simulink model "FluxObserverTest"  (R2026b)
settings: Solver=FixedStepDiscrete  StopTime=fluxTestCfg.Duration  FixedStep=fluxCfg.Ts
PostLoadFcn:
  | addpath(fullfile(fileparts(get_param(bdroot,'FileName')),'..','build_process'));initialize_flux_test(bdroot);
model workspace (MAT data in the model file):
  fluxCfg.Ts = 5e-05
  fluxCfg.Rs = 0.5
  fluxCfg.L = 0.001
  fluxCfg.Flux = 0.035
  fluxCfg.PolePairs = 4
  fluxCfg.LeakEnable = 1
  fluxCfg.LeakHz = 10
  fluxCfg.DcEnable = 1
  fluxCfg.DcHz = 3
  fluxCfg.FrequencyHz = 5
  fluxCfg.MinCompOmega = 20
  fluxCfg.FullCompOmega = 100
  fluxCfg.MaxCompGain = 4
  fluxCfg.MinFlux = 0.015
  fluxCfg.MaxFlux = 0.0525
  fluxCfg.MinOmega = 120
  fluxCfg.MaxResidual = 5
  fluxCfg.LeakA = 0.996863336985
  fluxCfg.LeakB = 4.99215423658e-05
  fluxCfg.DcA = 0.999057966197
  fluxCfg.FrequencyA = 0.998430436728
  fluxTestCfg.Duration = 1
  fluxTestCfg.ElectricalSpeed = 200
  fluxTestCfg.InitialAngle = 0.4
  fluxTestCfg.Id = -2
  fluxTestCfg.Iq = 2
  fluxTestCfg.Enable = 1
  fluxTestCfg.Reset = 0
  pllCfg.Ts = 5e-05
  pllCfg.NaturalFrequency = 40
  pllCfg.Damping = 0.707
  pllCfg.Kp = 355.376960974
  pllCfg.Ki = 63165.468167
  pllCfg.Kaw = 502.654824574
  pllCfg.OmegaMax = 1500
  pllCfg.MinMagnitude = 0.015
  pllCfg.LockError = 0.12
  pllCfg.LockSamples = 100
  pllCfg.Theta0 = 0
  pllCfg.Omega0 = 0
  testStim.time = []
  testStim.signals.values = [-4.24906479315 -4.31340004462 -4.37730395969 -4.44077014801 -4.50379226301 -4.56636400254 -4.62847910947 -4.69013137235 -4.75131462601 -4.81202275215 -4.87224968004 -4.93198938701 ... (180009 elements, 20001x9)]
  testStim.signals.dimensions = 9
libraries: FluxObserver x1
settings Model: Creator=24322  LastModifiedBy=24322

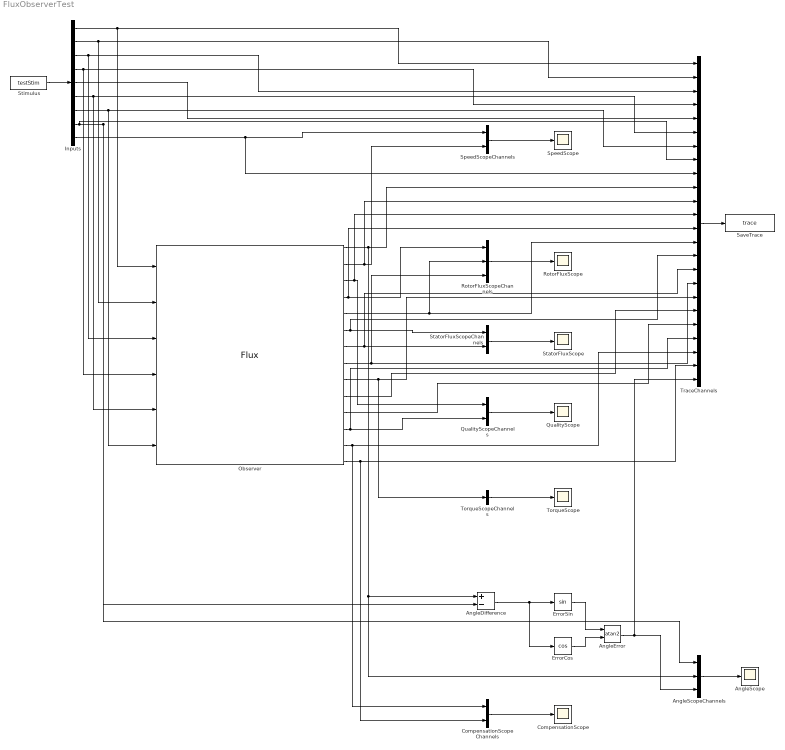
== system FluxObserverTest ==
  AngleDifference : Sum  Inputs=+-
  AngleError : Trigonometry  Operator=atan2
  AngleScope : Scope
  AngleScopeChannels : Mux  Inputs=3
  CompensationScope : Scope
  CompensationScopeChannels : Mux  Inputs=2
  ErrorCos : Trigonometry  Operator=cos
  ErrorSin : Trigonometry
  Inputs : Demux  Outputs=9
  Observer : FluxObserver/Flux  cfg=fluxCfg  trackerCfg=pllCfg
  QualityScope : Scope
  QualityScopeChannels : Mux  Inputs=2
  RotorFluxScope : Scope
  RotorFluxScopeChannels : Mux  Inputs=3
  SaveTrace : ToWorkspace  VariableName=trace  SaveFormat=Structure With Time  SampleTime=-1
  SpeedScope : Scope
  SpeedScopeChannels : Mux  Inputs=2
  StatorFluxScope : Scope
  StatorFluxScopeChannels : Mux  Inputs=2
  Stimulus : FromWorkspace  VariableName=testStim  SampleTime=fluxCfg.Ts  Interpolate=off  OutputAfterFinalValue=Holding final value
  TorqueScope : Scope
  TorqueScopeChannels : Mux  Inputs=1
  TraceChannels : Mux  Inputs=24
  wires:
  CompensationScopeChannels/1 -> CompensationScope/1
  QualityScopeChannels/1 -> QualityScope/1
  TorqueScopeChannels/1 -> TorqueScope/1
  StatorFluxScopeChannels/1 -> StatorFluxScope/1
  RotorFluxScopeChannels/1 -> RotorFluxScope/1
  SpeedScopeChannels/1 -> SpeedScope/1
  AngleScopeChannels/1 -> AngleScope/1
  Observer/14 -> TraceChannels/23, CompensationScopeChannels/2
  Observer/13 -> TraceChannels/22, CompensationScopeChannels/1
  Observer/12 -> QualityScopeChannels/2, TraceChannels/21
  Observer/11 -> TraceChannels/20
  Observer/10 -> TraceChannels/19
  Observer/9 -> TraceChannels/18, TorqueScopeChannels/1
  Observer/8 -> TraceChannels/17, RotorFluxScopeChannels/3
  Observer/7 -> StatorFluxScopeChannels/2, TraceChannels/16
  Observer/6 -> StatorFluxScopeChannels/1, TraceChannels/15
  Observer/5 -> TraceChannels/14, RotorFluxScopeChannels/2
  Observer/4 -> TraceChannels/13, RotorFluxScopeChannels/1
  Observer/3 -> TraceChannels/12, QualityScopeChannels/1
  Observer/2 -> TraceChannels/11, SpeedScopeChannels/2
  Inputs/9 -> SpeedScopeChannels/1, TraceChannels/9
  Inputs/5 -> TraceChannels/5
  Inputs/7 -> Observer/6, TraceChannels/7
  Inputs/6 -> Observer/5, TraceChannels/6
  Inputs/4 -> Observer/4, TraceChannels/4
  Inputs/3 -> Observer/3, TraceChannels/3
  Inputs/2 -> Observer/2, TraceChannels/2
  Inputs/1 -> Observer/1, TraceChannels/1
  TraceChannels/1 -> SaveTrace/1
  AngleError/1 -> TraceChannels/24, AngleScopeChannels/3
  ErrorCos/1 -> AngleError/2
  ErrorSin/1 -> AngleError/1
  AngleDifference/1 -> ErrorSin/1, ErrorCos/1
  Inputs/8 -> AngleDifference/2, AngleScopeChannels/1, TraceChannels/8
  Observer/1 -> AngleDifference/1, AngleScopeChannels/2, TraceChannels/10
  Stimulus/1 -> Inputs/1
